simulink model "Crazyflie_Sim_R2025b"  (R2025b)
settings: Solver=ode15s  StopTime=20  RelTol=1e-5
InitFcn:
  | Crazyflie_Param
values from neighbouring files (symbols this model uses):
  g = 9.80665    [Crazyflie_Param.m]
  Ix_drone = 2.934e-5    (= 2.934e-05)    [Crazyflie_Param.m]
  Iy_drone = 4.981e-5    (= 4.981e-05)    [Crazyflie_Param.m]
  Iz_drone = 7.646e-5    (= 7.646e-05)    [Crazyflie_Param.m]
  J = 1/12*m*(0.051^2+0.005^2)    (= 7.878e-08)    [Crazyflie_Param.m]
  kq = 0.006    [Crazyflie_Param.m]
  l1 = 4.445    [Crazyflie_Param.m]
  m = 0.00036    [Crazyflie_Param.m]
  m_drone = 0.04316    [Crazyflie_Param.m]
undefined symbols (not defined in the file or in its folder): sigbuilder_block, X, Y, Z
libraries: sm_lib x57, slpidlib x19, nesl_utility x18, fl_lib x9
(part 2 of 4)

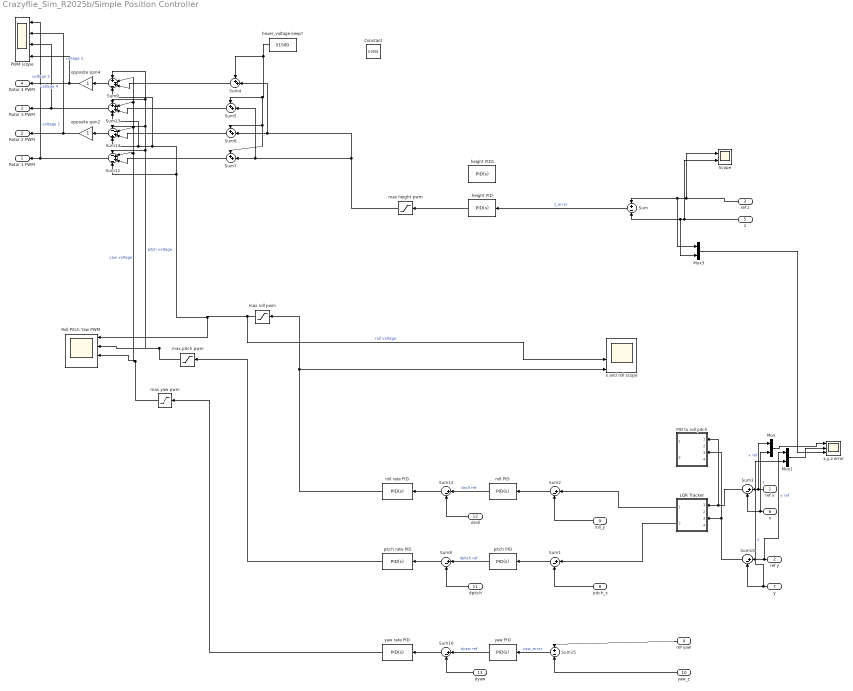
== system Crazyflie_Sim_R2025b/Simple Position Controller ==
  ref x : Inport
  ref y : Inport  Port=2
  ref z : Inport  Port=3
  ref yaw : Inport  Port=4
  z : Inport  Port=5
  x : Inport  Port=6
  y : Inport  Port=7
  pitch_x : Inport  Port=8
  roll_y : Inport  Port=9
  yaw_z : Inport  Port=10
  dpitch : Inport  Port=11
  droll : Inport  Port=12
  dyaw : Inport  Port=13
  Constant : Constant  Value=0.0001
  LQR Tracker : Subsystem
  Mux : Mux  Inputs=2
  Mux1 : Mux  Inputs=2
  Mux3 : Mux  Inputs=2
  PID to roll pitch : Subsystem
  PWM scope : Scope  NumInputPorts=4
      settings: ActiveDisplayYMinimum=30000  ActiveDisplayYMaximum=50000
  Roll Pitch Yaw PWM : Scope  NumInputPorts=4
      settings: ActiveDisplayYMinimum=-81918.75  ActiveDisplayYMaximum=81918.75
  Scope : Scope  NumInputPorts=2
      settings: ActiveDisplayYMinimum=-0.12883916669712672  ActiveDisplayYMaximum=1.1595525002741407  DataLoggingVariableName=ScopeData2
  Sum : Sum  Inputs=+-
  Sum{1..3,8,10,12,16} (7 alike) : Sum  Inputs=|+-
  Sum11 : Sum  Inputs=-++-
  Sum13 : Sum  Inputs=++++
  Sum14 : Sum  Inputs=--++
  Sum15 : Sum  Inputs=+-
  Sum{4..7} (4 alike) : Sum  Inputs=++|
  Sum9 : Sum  Inputs=+-+-
  height PID : slpidlib/PID Controller  Controller=PID  Form=Parallel  TimeDomain=Continuous-time  UseExternalTs=off  SampleTime=-1  IntegratorMethod=Forward Euler  FilterMethod=Forward Euler  ControllerParametersSource=internal  P=30000  I=100  UseKiTs=off  D=15000  UseExternalDerivativeSource=off  N=100  UseFilter=on  TunerSelectOption=Transfer Function Based (PID Tuner App)  ZeroCross=off  InitialConditionSource=internal  InitialConditionForIntegrator=0  InitialConditionForFilter=0  DifferentiatorICPrevScaledInput=0  ExternalReset=none  TrackingMode=off  Kt=1  LimitOutput=off  SatLimitsSource=internal  UpperSaturationLimit=inf  LowerSaturationLimit=-inf  LinearizeAsGain=on  AntiWindupMode=none  Kb=1  LimitIntegrator=off  UpperIntegratorSaturationLimit=inf  LowerIntegratorSaturationLimit=-inf  POutMin=[]  POutMax=[]  IOutMin=[]  IOutMax=[]  DOutMin=[]  DOutMax=[]  NOutMin=[]  NOutMax=[]  SumOutMin=[]  SumOutMax=[]  SaturationOutMin=[]  SaturationOutMax=[]  PParamMin=[]  PParamMax=[]  IParamMin=[]  IParamMax=[]  DParamMin=[]  DParamMax=[]  NParamMin=[]  NParamMax=[]  KbParamMin=[]  KbParamMax=[]  KtParamMin=[]  KtParamMax=[]  KbOutMin=[]  KbOutMax=[]  KtOutMin=[]  KtOutMax=[]  IntegratorOutMin=[]  IntegratorOutMax=[]  FilterOutMin=[]  FilterOutMax=[]  SumI1OutMin=[]  SumI1OutMax=[]  SumI2OutMin=[]  SumI2OutMax=[]  SumI3OutMin=[]  SumI3OutMax=[]  SumI4OutMin=[]  SumI4OutMax=[]  SumDOutMin=[]  SumDOutMax=[]  DifferentiatorOutMin=[]  DifferentiatorOutMax=[]  FilterDiffOutCoefMin=[]  FilterDiffOutCoefMax=[]  ReciprocalOutMin=[]  ReciprocalOutMax=[]  SumDenOutMin=[]  SumDenOutMax=[]  SumNumOutMin=[]  SumNumOutMax=[]  DivideOutMin=[]  DivideOutMax=[]  UdiffTsProdOutMin=[]  UdiffTsProdOutMax=[]  NTsProdOutMin=[]  NTsProdOutMax=[]  UintegralTsProdOutMin=[]  UintegralTsProdOutMax=[]  UngainTsProdOutMin=[]  UngainTsProdOutMax=[]  ClampingZeroOutDataTypeStr=Inherit: Inherit via back propagation  ClampingZeroOutMin=[]  ClampingZeroOutMax=[]  FilterDenConstantOutDataTypeStr=Inherit: Inherit via back propagation  FilterDenConstantOutMin=[]  FilterDenConstantOutMax=[]  PCopyOutDataTypeStr=Inherit: Inherit via back propagation  PCopyOutMin=[]  PCopyOutMax=[]  NCopyOutDataTypeStr=Inherit: Inherit via back propagation  NCopyOutMin=[]  NCopyOutMax=[]  IntegratorContinuousStateAttributes=''  IntegratorStateMustResolveToSignalObject=off  IntegratorRTWStateStorageClass=Auto  FilterContinuousStateAttributes=''  FilterStateMustResolveToSignalObject=off  FilterRTWStateStorageClass=Auto  ParallelPVariant=InternalParameters  IdealPVariant=Disabled  IVariant=InternalParameters  DVariant=InternalParameters  IntegratorVariant=Continuous  SatVariant=Disabled  AWVariant=Passthrough  PCopyVariant=Disabled  TRVariant=Disabled  FdbkBlocksVariant=Forward  IdealPFdbkVariant=Disabled  SatFdbkVariant=Disabled  DerivativeFilterVariant=ContFilter  NVariant=InternalParameters  NCopyVariant=Disabled  FilterICVariant=InternalICsFilter  IntegratorICVariant=InternalICs  ExternalResetVariant=Disabled  TRSumVariant=Passthrough  SumFdbkVariant=Disabled  SumVariant=Sum_PID  TsampFilterVariant=InternalTs  TsampNgainVariant=Passthrough  TsampIntegralVariant=Disabled_SignalSpec  ExternalSaturationOutDataTypeStr=Inherit: Same as second input  DerivativeSourceVariant=ErrorSignal  PreIntVariant=InternalPreInt
  height PID1 : slpidlib/PID Controller  Controller=PID  Form=Parallel  TimeDomain=Continuous-time  UseExternalTs=off  SampleTime=-1  IntegratorMethod=Forward Euler  FilterMethod=Forward Euler  ControllerParametersSource=internal  P=14649  I=0  UseKiTs=off  D=6252  UseExternalDerivativeSource=off  N=100  UseFilter=on  TunerSelectOption=Transfer Function Based (PID Tuner App)  InitialConditionSource=internal  InitialConditionForIntegrator=0  InitialConditionForFilter=0  DifferentiatorICPrevScaledInput=0  ExternalReset=none  TrackingMode=off  Kt=1  LimitOutput=off  SatLimitsSource=internal  UpperSaturationLimit=inf  LowerSaturationLimit=-inf  LinearizeAsGain=on  AntiWindupMode=none  Kb=1  LimitIntegrator=off  UpperIntegratorSaturationLimit=inf  LowerIntegratorSaturationLimit=-inf  POutMin=[]  POutMax=[]  IOutMin=[]  IOutMax=[]  DOutMin=[]  DOutMax=[]  NOutMin=[]  NOutMax=[]  SumOutMin=[]  SumOutMax=[]  SaturationOutMin=[]  SaturationOutMax=[]  PParamMin=[]  PParamMax=[]  IParamMin=[]  IParamMax=[]  DParamMin=[]  DParamMax=[]  NParamMin=[]  NParamMax=[]  KbParamMin=[]  KbParamMax=[]  KtParamMin=[]  KtParamMax=[]  KbOutMin=[]  KbOutMax=[]  KtOutMin=[]  KtOutMax=[]  IntegratorOutMin=[]  IntegratorOutMax=[]  FilterOutMin=[]  FilterOutMax=[]  SumI1OutMin=[]  SumI1OutMax=[]  SumI2OutMin=[]  SumI2OutMax=[]  SumI3OutMin=[]  SumI3OutMax=[]  SumI4OutMin=[]  SumI4OutMax=[]  SumDOutMin=[]  SumDOutMax=[]  DifferentiatorOutMin=[]  DifferentiatorOutMax=[]  FilterDiffOutCoefMin=[]  FilterDiffOutCoefMax=[]  ReciprocalOutMin=[]  ReciprocalOutMax=[]  SumDenOutMin=[]  SumDenOutMax=[]  SumNumOutMin=[]  SumNumOutMax=[]  DivideOutMin=[]  DivideOutMax=[]  UdiffTsProdOutMin=[]  UdiffTsProdOutMax=[]  NTsProdOutMin=[]  NTsProdOutMax=[]  UintegralTsProdOutMin=[]  UintegralTsProdOutMax=[]  UngainTsProdOutMin=[]  UngainTsProdOutMax=[]  ClampingZeroOutDataTypeStr=Inherit: Inherit via back propagation  ClampingZeroOutMin=[]  ClampingZeroOutMax=[]  FilterDenConstantOutDataTypeStr=Inherit: Inherit via back propagation  FilterDenConstantOutMin=[]  FilterDenConstantOutMax=[]  PCopyOutDataTypeStr=Inherit: Inherit via back propagation  PCopyOutMin=[]  PCopyOutMax=[]  NCopyOutDataTypeStr=Inherit: Inherit via back propagation  NCopyOutMin=[]  NCopyOutMax=[]  IntegratorContinuousStateAttributes=''  IntegratorStateMustResolveToSignalObject=off  IntegratorRTWStateStorageClass=Auto  FilterContinuousStateAttributes=''  FilterStateMustResolveToSignalObject=off  FilterRTWStateStorageClass=Auto  ParallelPVariant=InternalParameters  IdealPVariant=Disabled  IVariant=InternalParameters  DVariant=InternalParameters  IntegratorVariant=Continuous  SatVariant=Disabled  AWVariant=Passthrough  PCopyVariant=Disabled  TRVariant=Disabled  FdbkBlocksVariant=Forward  IdealPFdbkVariant=Disabled  SatFdbkVariant=Disabled  DerivativeFilterVariant=ContFilter  NVariant=InternalParameters  NCopyVariant=Disabled  FilterICVariant=InternalICsFilter  IntegratorICVariant=InternalICs  ExternalResetVariant=Disabled  TRSumVariant=Passthrough  SumFdbkVariant=Disabled  SumVariant=Sum_PID  TsampFilterVariant=InternalTs  TsampNgainVariant=Passthrough  TsampIntegralVariant=Disabled_SignalSpec  ExternalSaturationOutDataTypeStr=Inherit: Same as second input  DerivativeSourceVariant=ErrorSignal  PreIntVariant=InternalPreInt
  hover_voltage keep? : Constant  Value=51500
  max height pwm : Saturate  UpperLimit=30000  LowerLimit=-38000  ZeroCross=off
  max pitch pwm : Saturate  UpperLimit=10000  LowerLimit=-10000  ZeroCross=off
  max roll pwm : Saturate  UpperLimit=10000  LowerLimit=-10000  ZeroCross=off
  max yaw pwm : Saturate  UpperLimit=10000  LowerLimit=-10000  ZeroCross=off
  opposite spin2 : Gain
  opposite spin4 : Gain
  pitch PID : slpidlib/PID Controller  Controller=PID  Form=Parallel  TimeDomain=Continuous-time  UseExternalTs=off  SampleTime=-1  IntegratorMethod=Forward Euler  FilterMethod=Forward Euler  ControllerParametersSource=internal  P=6  I=3  UseKiTs=off  D=0  UseExternalDerivativeSource=off  N=100  UseFilter=on  TunerSelectOption=Transfer Function Based (PID Tuner App)  InitialConditionSource=internal  InitialConditionForIntegrator=0  InitialConditionForFilter=0  DifferentiatorICPrevScaledInput=0  ExternalReset=none  TrackingMode=off  Kt=1  LimitOutput=off  SatLimitsSource=internal  UpperSaturationLimit=inf  LowerSaturationLimit=-inf  LinearizeAsGain=on  AntiWindupMode=none  Kb=1  LimitIntegrator=off  UpperIntegratorSaturationLimit=inf  LowerIntegratorSaturationLimit=-inf  POutMin=[]  POutMax=[]  IOutMin=[]  IOutMax=[]  DOutMin=[]  DOutMax=[]  NOutMin=[]  NOutMax=[]  SumOutMin=[]  SumOutMax=[]  SaturationOutMin=[]  SaturationOutMax=[]  PParamMin=[]  PParamMax=[]  IParamMin=[]  IParamMax=[]  DParamMin=[]  DParamMax=[]  NParamMin=[]  NParamMax=[]  KbParamMin=[]  KbParamMax=[]  KtParamMin=[]  KtParamMax=[]  KbOutMin=[]  KbOutMax=[]  KtOutMin=[]  KtOutMax=[]  IntegratorOutMin=[]  IntegratorOutMax=[]  FilterOutMin=[]  FilterOutMax=[]  SumI1OutMin=[]  SumI1OutMax=[]  SumI2OutMin=[]  SumI2OutMax=[]  SumI3OutMin=[]  SumI3OutMax=[]  SumI4OutMin=[]  SumI4OutMax=[]  SumDOutMin=[]  SumDOutMax=[]  DifferentiatorOutMin=[]  DifferentiatorOutMax=[]  FilterDiffOutCoefMin=[]  FilterDiffOutCoefMax=[]  ReciprocalOutMin=[]  ReciprocalOutMax=[]  SumDenOutMin=[]  SumDenOutMax=[]  SumNumOutMin=[]  SumNumOutMax=[]  DivideOutMin=[]  DivideOutMax=[]  UdiffTsProdOutMin=[]  UdiffTsProdOutMax=[]  NTsProdOutMin=[]  NTsProdOutMax=[]  UintegralTsProdOutMin=[]  UintegralTsProdOutMax=[]  UngainTsProdOutMin=[]  UngainTsProdOutMax=[]  ClampingZeroOutDataTypeStr=Inherit: Inherit via back propagation  ClampingZeroOutMin=[]  ClampingZeroOutMax=[]  FilterDenConstantOutDataTypeStr=Inherit: Inherit via back propagation  FilterDenConstantOutMin=[]  FilterDenConstantOutMax=[]  PCopyOutDataTypeStr=Inherit: Inherit via back propagation  PCopyOutMin=[]  PCopyOutMax=[]  NCopyOutDataTypeStr=Inherit: Inherit via back propagation  NCopyOutMin=[]  NCopyOutMax=[]  IntegratorContinuousStateAttributes=''  IntegratorStateMustResolveToSignalObject=off  IntegratorRTWStateStorageClass=Auto  FilterContinuousStateAttributes=''  FilterStateMustResolveToSignalObject=off  FilterRTWStateStorageClass=Auto  ParallelPVariant=InternalParameters  IdealPVariant=Disabled  IVariant=InternalParameters  DVariant=InternalParameters  IntegratorVariant=Continuous  SatVariant=Disabled  AWVariant=Passthrough  PCopyVariant=Disabled  TRVariant=Disabled  FdbkBlocksVariant=Forward  IdealPFdbkVariant=Disabled  SatFdbkVariant=Disabled  DerivativeFilterVariant=ContFilter  NVariant=InternalParameters  NCopyVariant=Disabled  FilterICVariant=InternalICsFilter  IntegratorICVariant=InternalICs  ExternalResetVariant=Disabled  TRSumVariant=Passthrough  SumFdbkVariant=Disabled  SumVariant=Sum_PID  TsampFilterVariant=InternalTs  TsampNgainVariant=Passthrough  TsampIntegralVariant=Disabled_SignalSpec  ExternalSaturationOutDataTypeStr=Inherit: Same as second input  DerivativeSourceVariant=ErrorSignal  PreIntVariant=InternalPreInt
  pitch rate PID : slpidlib/PID Controller  Controller=PID  Form=Parallel  TimeDomain=Continuous-time  UseExternalTs=off  SampleTime=-1  IntegratorMethod=Forward Euler  FilterMethod=Forward Euler  ControllerParametersSource=internal  P=250*3.1  I=500*3.1  UseKiTs=off  D=2.5*3.1  UseExternalDerivativeSource=off  N=100  UseFilter=on  TunerSelectOption=Transfer Function Based (PID Tuner App)  InitialConditionSource=internal  InitialConditionForIntegrator=0  InitialConditionForFilter=0  DifferentiatorICPrevScaledInput=0  ExternalReset=none  TrackingMode=off  Kt=1  LimitOutput=off  SatLimitsSource=internal  UpperSaturationLimit=inf  LowerSaturationLimit=-inf  LinearizeAsGain=on  AntiWindupMode=none  Kb=1  LimitIntegrator=off  UpperIntegratorSaturationLimit=inf  LowerIntegratorSaturationLimit=-inf  POutMin=[]  POutMax=[]  IOutMin=[]  IOutMax=[]  DOutMin=[]  DOutMax=[]  NOutMin=[]  NOutMax=[]  SumOutMin=[]  SumOutMax=[]  SaturationOutMin=[]  SaturationOutMax=[]  PParamMin=[]  PParamMax=[]  IParamMin=[]  IParamMax=[]  DParamMin=[]  DParamMax=[]  NParamMin=[]  NParamMax=[]  KbParamMin=[]  KbParamMax=[]  KtParamMin=[]  KtParamMax=[]  KbOutMin=[]  KbOutMax=[]  KtOutMin=[]  KtOutMax=[]  IntegratorOutMin=[]  IntegratorOutMax=[]  FilterOutMin=[]  FilterOutMax=[]  SumI1OutMin=[]  SumI1OutMax=[]  SumI2OutMin=[]  SumI2OutMax=[]  SumI3OutMin=[]  SumI3OutMax=[]  SumI4OutMin=[]  SumI4OutMax=[]  SumDOutMin=[]  SumDOutMax=[]  DifferentiatorOutMin=[]  DifferentiatorOutMax=[]  FilterDiffOutCoefMin=[]  FilterDiffOutCoefMax=[]  ReciprocalOutMin=[]  ReciprocalOutMax=[]  SumDenOutMin=[]  SumDenOutMax=[]  SumNumOutMin=[]  SumNumOutMax=[]  DivideOutMin=[]  DivideOutMax=[]  UdiffTsProdOutMin=[]  UdiffTsProdOutMax=[]  NTsProdOutMin=[]  NTsProdOutMax=[]  UintegralTsProdOutMin=[]  UintegralTsProdOutMax=[]  UngainTsProdOutMin=[]  UngainTsProdOutMax=[]  ClampingZeroOutDataTypeStr=Inherit: Inherit via back propagation  ClampingZeroOutMin=[]  ClampingZeroOutMax=[]  FilterDenConstantOutDataTypeStr=Inherit: Inherit via back propagation  FilterDenConstantOutMin=[]  FilterDenConstantOutMax=[]  PCopyOutDataTypeStr=Inherit: Inherit via back propagation  PCopyOutMin=[]  PCopyOutMax=[]  NCopyOutDataTypeStr=Inherit: Inherit via back propagation  NCopyOutMin=[]  NCopyOutMax=[]  IntegratorContinuousStateAttributes=''  IntegratorStateMustResolveToSignalObject=off  IntegratorRTWStateStorageClass=Auto  FilterContinuousStateAttributes=''  FilterStateMustResolveToSignalObject=off  FilterRTWStateStorageClass=Auto  ParallelPVariant=InternalParameters  IdealPVariant=Disabled  IVariant=InternalParameters  DVariant=InternalParameters  IntegratorVariant=Continuous  SatVariant=Disabled  AWVariant=Passthrough  PCopyVariant=Disabled  TRVariant=Disabled  FdbkBlocksVariant=Forward  IdealPFdbkVariant=Disabled  SatFdbkVariant=Disabled  DerivativeFilterVariant=ContFilter  NVariant=InternalParameters  NCopyVariant=Disabled  FilterICVariant=InternalICsFilter  IntegratorICVariant=InternalICs  ExternalResetVariant=Disabled  TRSumVariant=Passthrough  SumFdbkVariant=Disabled  SumVariant=Sum_PID  TsampFilterVariant=InternalTs  TsampNgainVariant=Passthrough  TsampIntegralVariant=Disabled_SignalSpec  ExternalSaturationOutDataTypeStr=Inherit: Same as second input  DerivativeSourceVariant=ErrorSignal  PreIntVariant=InternalPreInt
  roll PID : slpidlib/PID Controller  Controller=PID  Form=Parallel  TimeDomain=Continuous-time  UseExternalTs=off  SampleTime=-1  IntegratorMethod=Forward Euler  FilterMethod=Forward Euler  ControllerParametersSource=internal  P=6  I=3  UseKiTs=off  D=0  UseExternalDerivativeSource=off  N=100  UseFilter=on  TunerSelectOption=Transfer Function Based (PID Tuner App)  InitialConditionSource=internal  InitialConditionForIntegrator=0  InitialConditionForFilter=0  DifferentiatorICPrevScaledInput=0  ExternalReset=none  TrackingMode=off  Kt=1  LimitOutput=off  SatLimitsSource=internal  UpperSaturationLimit=inf  LowerSaturationLimit=-inf  LinearizeAsGain=on  AntiWindupMode=none  Kb=1  LimitIntegrator=off  UpperIntegratorSaturationLimit=inf  LowerIntegratorSaturationLimit=-inf  POutMin=[]  POutMax=[]  IOutMin=[]  IOutMax=[]  DOutMin=[]  DOutMax=[]  NOutMin=[]  NOutMax=[]  SumOutMin=[]  SumOutMax=[]  SaturationOutMin=[]  SaturationOutMax=[]  PParamMin=[]  PParamMax=[]  IParamMin=[]  IParamMax=[]  DParamMin=[]  DParamMax=[]  NParamMin=[]  NParamMax=[]  KbParamMin=[]  KbParamMax=[]  KtParamMin=[]  KtParamMax=[]  KbOutMin=[]  KbOutMax=[]  KtOutMin=[]  KtOutMax=[]  IntegratorOutMin=[]  IntegratorOutMax=[]  FilterOutMin=[]  FilterOutMax=[]  SumI1OutMin=[]  SumI1OutMax=[]  SumI2OutMin=[]  SumI2OutMax=[]  SumI3OutMin=[]  SumI3OutMax=[]  SumI4OutMin=[]  SumI4OutMax=[]  SumDOutMin=[]  SumDOutMax=[]  DifferentiatorOutMin=[]  DifferentiatorOutMax=[]  FilterDiffOutCoefMin=[]  FilterDiffOutCoefMax=[]  ReciprocalOutMin=[]  ReciprocalOutMax=[]  SumDenOutMin=[]  SumDenOutMax=[]  SumNumOutMin=[]  SumNumOutMax=[]  DivideOutMin=[]  DivideOutMax=[]  UdiffTsProdOutMin=[]  UdiffTsProdOutMax=[]  NTsProdOutMin=[]  NTsProdOutMax=[]  UintegralTsProdOutMin=[]  UintegralTsProdOutMax=[]  UngainTsProdOutMin=[]  UngainTsProdOutMax=[]  ClampingZeroOutDataTypeStr=Inherit: Inherit via back propagation  ClampingZeroOutMin=[]  ClampingZeroOutMax=[]  FilterDenConstantOutDataTypeStr=Inherit: Inherit via back propagation  FilterDenConstantOutMin=[]  FilterDenConstantOutMax=[]  PCopyOutDataTypeStr=Inherit: Inherit via back propagation  PCopyOutMin=[]  PCopyOutMax=[]  NCopyOutDataTypeStr=Inherit: Inherit via back propagation  NCopyOutMin=[]  NCopyOutMax=[]  IntegratorContinuousStateAttributes=''  IntegratorStateMustResolveToSignalObject=off  IntegratorRTWStateStorageClass=Auto  FilterContinuousStateAttributes=''  FilterStateMustResolveToSignalObject=off  FilterRTWStateStorageClass=Auto  ParallelPVariant=InternalParameters  IdealPVariant=Disabled  IVariant=InternalParameters  DVariant=InternalParameters  IntegratorVariant=Continuous  SatVariant=Disabled  AWVariant=Passthrough  PCopyVariant=Disabled  TRVariant=Disabled  FdbkBlocksVariant=Forward  IdealPFdbkVariant=Disabled  SatFdbkVariant=Disabled  DerivativeFilterVariant=ContFilter  NVariant=InternalParameters  NCopyVariant=Disabled  FilterICVariant=InternalICsFilter  IntegratorICVariant=InternalICs  ExternalResetVariant=Disabled  TRSumVariant=Passthrough  SumFdbkVariant=Disabled  SumVariant=Sum_PID  TsampFilterVariant=InternalTs  TsampNgainVariant=Passthrough  TsampIntegralVariant=Disabled_SignalSpec  ExternalSaturationOutDataTypeStr=Inherit: Same as second input  DerivativeSourceVariant=ErrorSignal  PreIntVariant=InternalPreInt
  roll rate PID : slpidlib/PID Controller  Controller=PID  Form=Parallel  TimeDomain=Continuous-time  UseExternalTs=off  SampleTime=-1  IntegratorMethod=Forward Euler  FilterMethod=Forward Euler  ControllerParametersSource=internal  P=250*3.1  I=500*3.1  UseKiTs=off  D=2.5*3.1  UseExternalDerivativeSource=off  N=100  UseFilter=on  TunerSelectOption=Transfer Function Based (PID Tuner App)  InitialConditionSource=internal  InitialConditionForIntegrator=0  InitialConditionForFilter=0  DifferentiatorICPrevScaledInput=0  ExternalReset=none  TrackingMode=off  Kt=1  LimitOutput=off  SatLimitsSource=internal  UpperSaturationLimit=inf  LowerSaturationLimit=-inf  LinearizeAsGain=on  AntiWindupMode=none  Kb=1  LimitIntegrator=off  UpperIntegratorSaturationLimit=inf  LowerIntegratorSaturationLimit=-inf  POutMin=[]  POutMax=[]  IOutMin=[]  IOutMax=[]  DOutMin=[]  DOutMax=[]  NOutMin=[]  NOutMax=[]  SumOutMin=[]  SumOutMax=[]  SaturationOutMin=[]  SaturationOutMax=[]  PParamMin=[]  PParamMax=[]  IParamMin=[]  IParamMax=[]  DParamMin=[]  DParamMax=[]  NParamMin=[]  NParamMax=[]  KbParamMin=[]  KbParamMax=[]  KtParamMin=[]  KtParamMax=[]  KbOutMin=[]  KbOutMax=[]  KtOutMin=[]  KtOutMax=[]  IntegratorOutMin=[]  IntegratorOutMax=[]  FilterOutMin=[]  FilterOutMax=[]  SumI1OutMin=[]  SumI1OutMax=[]  SumI2OutMin=[]  SumI2OutMax=[]  SumI3OutMin=[]  SumI3OutMax=[]  SumI4OutMin=[]  SumI4OutMax=[]  SumDOutMin=[]  SumDOutMax=[]  DifferentiatorOutMin=[]  DifferentiatorOutMax=[]  FilterDiffOutCoefMin=[]  FilterDiffOutCoefMax=[]  ReciprocalOutMin=[]  ReciprocalOutMax=[]  SumDenOutMin=[]  SumDenOutMax=[]  SumNumOutMin=[]  SumNumOutMax=[]  DivideOutMin=[]  DivideOutMax=[]  UdiffTsProdOutMin=[]  UdiffTsProdOutMax=[]  NTsProdOutMin=[]  NTsProdOutMax=[]  UintegralTsProdOutMin=[]  UintegralTsProdOutMax=[]  UngainTsProdOutMin=[]  UngainTsProdOutMax=[]  ClampingZeroOutDataTypeStr=Inherit: Inherit via back propagation  ClampingZeroOutMin=[]  ClampingZeroOutMax=[]  FilterDenConstantOutDataTypeStr=Inherit: Inherit via back propagation  FilterDenConstantOutMin=[]  FilterDenConstantOutMax=[]  PCopyOutDataTypeStr=Inherit: Inherit via back propagation  PCopyOutMin=[]  PCopyOutMax=[]  NCopyOutDataTypeStr=Inherit: Inherit via back propagation  NCopyOutMin=[]  NCopyOutMax=[]  IntegratorContinuousStateAttributes=''  IntegratorStateMustResolveToSignalObject=off  IntegratorRTWStateStorageClass=Auto  FilterContinuousStateAttributes=''  FilterStateMustResolveToSignalObject=off  FilterRTWStateStorageClass=Auto  ParallelPVariant=InternalParameters  IdealPVariant=Disabled  IVariant=InternalParameters  DVariant=InternalParameters  IntegratorVariant=Continuous  SatVariant=Disabled  AWVariant=Passthrough  PCopyVariant=Disabled  TRVariant=Disabled  FdbkBlocksVariant=Forward  IdealPFdbkVariant=Disabled  SatFdbkVariant=Disabled  DerivativeFilterVariant=ContFilter  NVariant=InternalParameters  NCopyVariant=Disabled  FilterICVariant=InternalICsFilter  IntegratorICVariant=InternalICs  ExternalResetVariant=Disabled  TRSumVariant=Passthrough  SumFdbkVariant=Disabled  SumVariant=Sum_PID  TsampFilterVariant=InternalTs  TsampNgainVariant=Passthrough  TsampIntegralVariant=Disabled_SignalSpec  ExternalSaturationOutDataTypeStr=Inherit: Same as second input  DerivativeSourceVariant=ErrorSignal  PreIntVariant=InternalPreInt
  "x and roll scope " : Scope  NumInputPorts=4
      settings: ActiveDisplayYMinimum=-11.1433  ActiveDisplayYMaximum=1.32628  DataLoggingVariableName=ScopeData3
  x,y,z error : Scope  NumInputPorts=3
      settings: ActiveDisplayYMinimum=-0.13989491710179006  ActiveDisplayYMaximum=1.25875136013476  DataLoggingVariableName=ScopeData2
  yaw PID : slpidlib/PID Controller  Controller=PID  Form=Parallel  TimeDomain=Continuous-time  UseExternalTs=off  SampleTime=-1  IntegratorMethod=Forward Euler  FilterMethod=Forward Euler  ControllerParametersSource=internal  P=6  I=1  UseKiTs=off  D=0.35  UseExternalDerivativeSource=off  N=100  UseFilter=on  TunerSelectOption=Transfer Function Based (PID Tuner App)  InitialConditionSource=internal  InitialConditionForIntegrator=0  InitialConditionForFilter=0  DifferentiatorICPrevScaledInput=0  ExternalReset=none  TrackingMode=off  Kt=1  LimitOutput=off  SatLimitsSource=internal  UpperSaturationLimit=inf  LowerSaturationLimit=-inf  LinearizeAsGain=on  AntiWindupMode=none  Kb=1  LimitIntegrator=off  UpperIntegratorSaturationLimit=inf  LowerIntegratorSaturationLimit=-inf  POutMin=[]  POutMax=[]  IOutMin=[]  IOutMax=[]  DOutMin=[]  DOutMax=[]  NOutMin=[]  NOutMax=[]  SumOutMin=[]  SumOutMax=[]  SaturationOutMin=[]  SaturationOutMax=[]  PParamMin=[]  PParamMax=[]  IParamMin=[]  IParamMax=[]  DParamMin=[]  DParamMax=[]  NParamMin=[]  NParamMax=[]  KbParamMin=[]  KbParamMax=[]  KtParamMin=[]  KtParamMax=[]  KbOutMin=[]  KbOutMax=[]  KtOutMin=[]  KtOutMax=[]  IntegratorOutMin=[]  IntegratorOutMax=[]  FilterOutMin=[]  FilterOutMax=[]  SumI1OutMin=[]  SumI1OutMax=[]  SumI2OutMin=[]  SumI2OutMax=[]  SumI3OutMin=[]  SumI3OutMax=[]  SumI4OutMin=[]  SumI4OutMax=[]  SumDOutMin=[]  SumDOutMax=[]  DifferentiatorOutMin=[]  DifferentiatorOutMax=[]  FilterDiffOutCoefMin=[]  FilterDiffOutCoefMax=[]  ReciprocalOutMin=[]  ReciprocalOutMax=[]  SumDenOutMin=[]  SumDenOutMax=[]  SumNumOutMin=[]  SumNumOutMax=[]  DivideOutMin=[]  DivideOutMax=[]  UdiffTsProdOutMin=[]  UdiffTsProdOutMax=[]  NTsProdOutMin=[]  NTsProdOutMax=[]  UintegralTsProdOutMin=[]  UintegralTsProdOutMax=[]  UngainTsProdOutMin=[]  UngainTsProdOutMax=[]  ClampingZeroOutDataTypeStr=Inherit: Inherit via back propagation  ClampingZeroOutMin=[]  ClampingZeroOutMax=[]  FilterDenConstantOutDataTypeStr=Inherit: Inherit via back propagation  FilterDenConstantOutMin=[]  FilterDenConstantOutMax=[]  PCopyOutDataTypeStr=Inherit: Inherit via back propagation  PCopyOutMin=[]  PCopyOutMax=[]  NCopyOutDataTypeStr=Inherit: Inherit via back propagation  NCopyOutMin=[]  NCopyOutMax=[]  IntegratorContinuousStateAttributes=''  IntegratorStateMustResolveToSignalObject=off  IntegratorRTWStateStorageClass=Auto  FilterContinuousStateAttributes=''  FilterStateMustResolveToSignalObject=off  FilterRTWStateStorageClass=Auto  ParallelPVariant=InternalParameters  IdealPVariant=Disabled  IVariant=InternalParameters  DVariant=InternalParameters  IntegratorVariant=Continuous  SatVariant=Disabled  AWVariant=Passthrough  PCopyVariant=Disabled  TRVariant=Disabled  FdbkBlocksVariant=Forward  IdealPFdbkVariant=Disabled  SatFdbkVariant=Disabled  DerivativeFilterVariant=ContFilter  NVariant=InternalParameters  NCopyVariant=Disabled  FilterICVariant=InternalICsFilter  IntegratorICVariant=InternalICs  ExternalResetVariant=Disabled  TRSumVariant=Passthrough  SumFdbkVariant=Disabled  SumVariant=Sum_PID  TsampFilterVariant=InternalTs  TsampNgainVariant=Passthrough  TsampIntegralVariant=Disabled_SignalSpec  ExternalSaturationOutDataTypeStr=Inherit: Same as second input  DerivativeSourceVariant=ErrorSignal  PreIntVariant=InternalPreInt
  yaw rate PID : slpidlib/PID Controller  Controller=PID  Form=Parallel  TimeDomain=Continuous-time  UseExternalTs=off  SampleTime=-1  IntegratorMethod=Forward Euler  FilterMethod=Forward Euler  ControllerParametersSource=internal  P=120*3.1  I=16.7*3.1  UseKiTs=off  D=0  UseExternalDerivativeSource=off  N=100  UseFilter=on  TunerSelectOption=Transfer Function Based (PID Tuner App)  InitialConditionSource=internal  InitialConditionForIntegrator=0  InitialConditionForFilter=0  DifferentiatorICPrevScaledInput=0  ExternalReset=none  TrackingMode=off  Kt=1  LimitOutput=off  SatLimitsSource=internal  UpperSaturationLimit=inf  LowerSaturationLimit=-inf  LinearizeAsGain=on  AntiWindupMode=none  Kb=1  LimitIntegrator=off  UpperIntegratorSaturationLimit=inf  LowerIntegratorSaturationLimit=-inf  POutMin=[]  POutMax=[]  IOutMin=[]  IOutMax=[]  DOutMin=[]  DOutMax=[]  NOutMin=[]  NOutMax=[]  SumOutMin=[]  SumOutMax=[]  SaturationOutMin=[]  SaturationOutMax=[]  PParamMin=[]  PParamMax=[]  IParamMin=[]  IParamMax=[]  DParamMin=[]  DParamMax=[]  NParamMin=[]  NParamMax=[]  KbParamMin=[]  KbParamMax=[]  KtParamMin=[]  KtParamMax=[]  KbOutMin=[]  KbOutMax=[]  KtOutMin=[]  KtOutMax=[]  IntegratorOutMin=[]  IntegratorOutMax=[]  FilterOutMin=[]  FilterOutMax=[]  SumI1OutMin=[]  SumI1OutMax=[]  SumI2OutMin=[]  SumI2OutMax=[]  SumI3OutMin=[]  SumI3OutMax=[]  SumI4OutMin=[]  SumI4OutMax=[]  SumDOutMin=[]  SumDOutMax=[]  DifferentiatorOutMin=[]  DifferentiatorOutMax=[]  FilterDiffOutCoefMin=[]  FilterDiffOutCoefMax=[]  ReciprocalOutMin=[]  ReciprocalOutMax=[]  SumDenOutMin=[]  SumDenOutMax=[]  SumNumOutMin=[]  SumNumOutMax=[]  DivideOutMin=[]  DivideOutMax=[]  UdiffTsProdOutMin=[]  UdiffTsProdOutMax=[]  NTsProdOutMin=[]  NTsProdOutMax=[]  UintegralTsProdOutMin=[]  UintegralTsProdOutMax=[]  UngainTsProdOutMin=[]  UngainTsProdOutMax=[]  ClampingZeroOutDataTypeStr=Inherit: Inherit via back propagation  ClampingZeroOutMin=[]  ClampingZeroOutMax=[]  FilterDenConstantOutDataTypeStr=Inherit: Inherit via back propagation  FilterDenConstantOutMin=[]  FilterDenConstantOutMax=[]  PCopyOutDataTypeStr=Inherit: Inherit via back propagation  PCopyOutMin=[]  PCopyOutMax=[]  NCopyOutDataTypeStr=Inherit: Inherit via back propagation  NCopyOutMin=[]  NCopyOutMax=[]  IntegratorContinuousStateAttributes=''  IntegratorStateMustResolveToSignalObject=off  IntegratorRTWStateStorageClass=Auto  FilterContinuousStateAttributes=''  FilterStateMustResolveToSignalObject=off  FilterRTWStateStorageClass=Auto  ParallelPVariant=InternalParameters  IdealPVariant=Disabled  IVariant=InternalParameters  DVariant=InternalParameters  IntegratorVariant=Continuous  SatVariant=Disabled  AWVariant=Passthrough  PCopyVariant=Disabled  TRVariant=Disabled  FdbkBlocksVariant=Forward  IdealPFdbkVariant=Disabled  SatFdbkVariant=Disabled  DerivativeFilterVariant=ContFilter  NVariant=InternalParameters  NCopyVariant=Disabled  FilterICVariant=InternalICsFilter  IntegratorICVariant=InternalICs  ExternalResetVariant=Disabled  TRSumVariant=Passthrough  SumFdbkVariant=Disabled  SumVariant=Sum_PID  TsampFilterVariant=InternalTs  TsampNgainVariant=Passthrough  TsampIntegralVariant=Disabled_SignalSpec  ExternalSaturationOutDataTypeStr=Inherit: Same as second input  DerivativeSourceVariant=ErrorSignal  PreIntVariant=InternalPreInt
  Rotor 1 PWM : Outport
  Rotor 2 PWM : Outport  Port=2
  Rotor 3 PWM : Outport  Port=3
  Rotor 4 PWM : Outport  Port=4
  wires:
  hover_voltage keep?/1 -> Sum4/1, Sum7/1, Sum6/1, Sum5/1
  Sum13/1 -> PWM scope/3, Rotor 3 PWM/1  "voltage 3"
  Sum11/1 -> Rotor 1 PWM/1, PWM scope/1  "voltage 1"
  Sum4/1 -> Sum9/3
  Sum6/1 -> Sum14/3
  opposite spin4/1 -> Rotor 4 PWM/1, PWM scope/4  "voltage 4"
  opposite spin2/1 -> PWM scope/2, Rotor 2 PWM/1  "voltage 2"
  ref z/1 -> Mux3/1, Sum/1, Scope/1
  z/1 -> Mux3/2, Sum/2, Scope/2
  Sum/1 -> height PID/1  "z_error"
  max roll pwm/1 -> Sum11/4, Sum14/4, Sum13/4, Sum9/4, Roll Pitch Yaw PWM/1, "x and roll scope "/3  "roll voltage"
  roll PID/1 -> Sum12/1  "droll ref"
  droll/1 -> Sum12/2
  Sum12/1 -> roll rate PID/1
  roll rate PID/1 -> max roll pwm/1, "x and roll scope "/4
  Sum8/1 -> pitch rate PID/1
  dpitch/1 -> Sum8/2
  pitch PID/1 -> Sum8/1  "dpitch ref"
  Sum5/1 -> Sum13/3
  Sum14/1 -> opposite spin2/1
  Sum9/1 -> opposite spin4/1
  Sum7/1 -> Sum11/3
  pitch rate PID/1 -> max pitch pwm/1
  max pitch pwm/1 -> Sum11/1, Sum14/1, Sum13/1, Sum9/1, Roll Pitch Yaw PWM/2  "pitch voltage"
  yaw rate PID/1 -> max yaw pwm/1
  ref yaw/1 -> Sum15/1
  yaw_z/1 -> Sum15/2
  Sum15/1 -> yaw PID/1  "yaw_error"
  yaw PID/1 -> Sum16/1  "dyaw ref"
  dyaw/1 -> Sum16/2
  Sum16/1 -> yaw rate PID/1
  max yaw pwm/1 -> Sum11/2, Sum14/2, Sum13/2, Sum9/2, Roll Pitch Yaw PWM/3  "yaw voltage"
  height PID/1 -> max height pwm/1
  Sum1/1 -> pitch PID/1
  pitch_x/1 -> Sum1/2
  Sum2/1 -> roll PID/1
  roll_y/1 -> Sum2/2
  ref x/1 -> Mux/1, Sum3/1  "x ref"
  x/1 -> Mux/2, Sum3/2  "x"
  ref y/1 -> Mux1/1, Sum10/1  "y ref"
  y/1 -> Mux1/2, Sum10/2  "y"
  Sum10/1 -> LQR Tracker/3(y error), PID to roll pitch/3(y error)
  Sum3/1 -> PID to roll pitch/1(x error), LQR Tracker/1(x error)
  LQR Tracker/1(roll ref) -> Sum2/1
  LQR Tracker/2(pitch ref) -> Sum1/1
  Mux/1 -> x,y,z error/1
  Mux1/1 -> x,y,z error/2
  max height pwm/1 -> Sum7/2, Sum5/2, Sum6/2, Sum4/2
  Mux3/1 -> x,y,z error/3

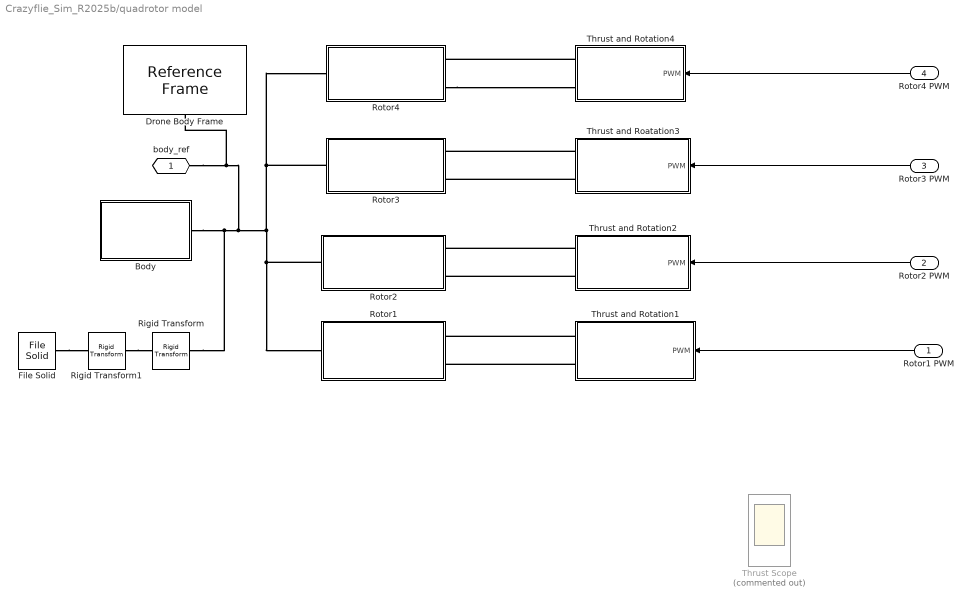
== system Crazyflie_Sim_R2025b/quadrotor model ==
  Rotor1 PWM : Inport
  Rotor2 PWM : Inport  Port=2
  Rotor3 PWM : Inport  Port=3
  Rotor4 PWM : Inport  Port=4
  Body : Subsystem
  Drone Body Frame : sm_lib/Frames and Transforms/Reference Frame
  File Solid : sm_lib/Body Elements/File Solid  ExtGeomFileName=C:\Users\lapsi\Documents\Work\Assignments\24-774\Project\CAD\Modified Crazyflie.step  UnitType=Custom  ExtGeomFileUnits=mm  StepReaderType=HEX  ExportConvexHullGeometry=off  InertiaType=PointMass  BasedOnType=DensityFromFile  Density=1000  DensityUnits=kg/m^3  Mass=0  MassUnits=kg  CenterOfMass=[0 0 0]  CenterOfMassUnits=m  MomentsOfInertia=[1 1 1]  MomentsOfInertiaUnits=kg*m^2  ProductsOfInertia=[0 0 0]  ProductsOfInertiaUnits=kg*m^2  GraphicType=FromGeometry  MarkerShape=Sphere  MarkerSize=10  GraphicVisPropType=AdvancedVisualProperties  GraphicDiffuseColor=[0.5 0.5 0.5]  GraphicOpacity=1  GraphicSpecularColor=[0.5 0.5 0.5 1.0]  GraphicAmbientColor=[0.15 0.15 0.15 1.0]  GraphicEmissiveColor=[0.0 0.0 0.0 1.0]  GraphicShininess=75  DoExposeReferenceFrame=on  SerializedFrames=<Frames/>
  Rigid Transform : sm_lib/Frames and Transforms/Rigid Transform  RotationMethod=StandardAxis  FollAlignAxisA=+X  BaseAlignAxisA=+Y  FollAlignAxisB=+Y  BaseAlignAxisB=+Z  RotationStandardAxis=+Z  RotationAngle=45  RotationAngleUnits=deg  RotationArbitraryAxis=[0 0 1]  RotationSequenceAxes=FollowerAxes  RotationSequence=XYX  RotationSequenceAngles=[0 0 0]  RotationSequenceAnglesUnits=deg  RotationMatrix=[1 0 0;0 1 0;0 0 1]  Quaternion=[1 0 0 0]  TranslationMethod=None  TranslationCartesianOffset=[0 0 0]  TranslationCartesianOffsetUnits=m  TranslationStandardAxis=+Z  TranslationStandardOffset=0  TranslationStandardOffsetUnits=m  TranslationROffset=0  TranslationROffsetUnits=m  TranslationThetaOffset=0  TranslationThetaOffsetUnits=deg  TranslationZOffset=0  TranslationZOffsetUnits=m
  Rigid Transform1 : sm_lib/Frames and Transforms/Rigid Transform  RotationMethod=StandardAxis  FollAlignAxisA=+X  BaseAlignAxisA=+Y  FollAlignAxisB=+Y  BaseAlignAxisB=+Z  RotationStandardAxis=+X  RotationAngle=180  RotationAngleUnits=deg  RotationArbitraryAxis=[0 0 1]  RotationSequenceAxes=FollowerAxes  RotationSequence=XYX  RotationSequenceAngles=[0 0 0]  RotationSequenceAnglesUnits=deg  RotationMatrix=[1 0 0;0 1 0;0 0 1]  Quaternion=[1 0 0 0]  TranslationMethod=None  TranslationCartesianOffset=[0 0 0]  TranslationCartesianOffsetUnits=m  TranslationStandardAxis=+Z  TranslationStandardOffset=0  TranslationStandardOffsetUnits=m  TranslationROffset=0  TranslationROffsetUnits=m  TranslationThetaOffset=0  TranslationThetaOffsetUnits=deg  TranslationZOffset=0  TranslationZOffsetUnits=m
  Rotor1 : Subsystem
  Rotor2 : Subsystem
  Rotor3 : Subsystem
  Rotor4 : Subsystem
  Thrust Scope : Scope  Commented=on  NumInputPorts=4
      settings: ActiveDisplayYMinimum=-1  ActiveDisplayYMaximum=1  DataLoggingVariableName=ScopeData2
  Thrust and Roatation3 : Subsystem
  Thrust and Rotation1 : Subsystem
  Thrust and Rotation2 : Subsystem
  Thrust and Rotation4 : Subsystem
  body_ref : PMIOPort  Side=Right
  wires:
  Rotor1 PWM/1 -> Thrust and Rotation1/1(PWM)
  Rotor2 PWM/1 -> Thrust and Rotation2/1(PWM)
  Rotor3 PWM/1 -> Thrust and Roatation3/1(PWM)
  Rotor4 PWM/1 -> Thrust and Rotation4/1(PWM)
  connections:
  Body/RConn1 -- Rigid Transform/RConn1 -- Rotor1/RConn1 -- Rotor2/LConn1 -- Rotor3/LConn1 -- Rotor4/LConn1 -- body_ref/RConn1 -- Drone Body Frame/RConn1
  Thrust and Rotation1/RConn1 -- Rotor1/LConn1
  Thrust and Rotation2/RConn1 -- Rotor2/RConn1
  Thrust and Rotation2/RConn2 -- Rotor2/RConn2
  Thrust and Roatation3/RConn1 -- Rotor3/RConn1
  Thrust and Rotation4/RConn1 -- Rotor4/RConn1
  File Solid/RConn1 -- Rigid Transform1/LConn1
  Rigid Transform1/RConn1 -- Rigid Transform/LConn1
  Thrust and Rotation1/RConn2 -- Rotor1/LConn2
  Thrust and Roatation3/RConn2 -- Rotor3/RConn2
  Rotor4/RConn2 -- Thrust and Rotation4/RConn2

== system Crazyflie_Sim_R2025b/6dof joint/Drone Reference Frame z-down,  + ==
  x +90 : sm_lib/Frames and Transforms/Rigid Transform  RotationMethod=StandardAxis  FollAlignAxisA=+X  BaseAlignAxisA=+Y  FollAlignAxisB=+Y  BaseAlignAxisB=+Z  RotationStandardAxis=+X  RotationAngle=90  RotationAngleUnits=deg  RotationArbitraryAxis=[0 0 1]  RotationSequenceAxes=FollowerAxes  RotationSequence=XYX  RotationSequenceAngles=[0 0 0]  RotationSequenceAnglesUnits=deg  RotationMatrix=[1 0 0; 0 1 0; 0 0 1]  Quaternion=[1 0 0 0]  TranslationMethod=None  TranslationCartesianOffset=[0 0 0]  TranslationCartesianOffsetUnits=m  TranslationStandardAxis=+Z  TranslationStandardOffset=0  TranslationStandardOffsetUnits=m  TranslationROffset=0  TranslationROffsetUnits=m  TranslationThetaOffset=0  TranslationThetaOffsetUnits=deg  TranslationZOffset=0  TranslationZOffsetUnits=m
  y -90 : sm_lib/Frames and Transforms/Rigid Transform  RotationMethod=StandardAxis  FollAlignAxisA=+X  BaseAlignAxisA=+Y  FollAlignAxisB=+Y  BaseAlignAxisB=+Z  RotationStandardAxis=+Y  RotationAngle=-90  RotationAngleUnits=deg  RotationArbitraryAxis=[0 0 1]  RotationSequenceAxes=FollowerAxes  RotationSequence=XYX  RotationSequenceAngles=[0 0 0]  RotationSequenceAnglesUnits=deg  RotationMatrix=[1 0 0; 0 1 0; 0 0 1]  Quaternion=[1 0 0 0]  TranslationMethod=None  TranslationCartesianOffset=[0 0 0]  TranslationCartesianOffsetUnits=m  TranslationStandardAxis=+Z  TranslationStandardOffset=0  TranslationStandardOffsetUnits=m  TranslationROffset=0  TranslationROffsetUnits=m  TranslationThetaOffset=0  TranslationThetaOffsetUnits=deg  TranslationZOffset=0  TranslationZOffsetUnits=m
  z-down : sm_lib/Frames and Transforms/Rigid Transform  RotationMethod=StandardAxis  FollAlignAxisA=+X  BaseAlignAxisA=+Y  FollAlignAxisB=+Y  BaseAlignAxisB=+Z  RotationStandardAxis=+X  RotationAngle=180  RotationAngleUnits=deg  RotationArbitraryAxis=[0 0 1]  RotationSequenceAxes=FollowerAxes  RotationSequence=XYX  RotationSequenceAngles=[0 0 0]  RotationSequenceAnglesUnits=deg  RotationMatrix=[1 0 0; 0 1 0; 0 0 1]  Quaternion=[1 0 0 0]  TranslationMethod=None  TranslationCartesianOffset=[0 0 0]  TranslationCartesianOffsetUnits=m  TranslationStandardAxis=+Z  TranslationStandardOffset=0  TranslationStandardOffsetUnits=m  TranslationROffset=0  TranslationROffsetUnits=m  TranslationThetaOffset=0  TranslationThetaOffsetUnits=deg  TranslationZOffset=0  TranslationZOffsetUnits=m
  Conn1 : PMIOPort  Side=Right
  Conn2 : PMIOPort  Port=2  Side=Left
  connections:
  Conn1/RConn1 -- z-down/RConn1
  y -90/RConn1 -- x +90/LConn1
  x +90/RConn1 -- z-down/LConn1
  Conn2/RConn1 -- y -90/LConn1

== system Crazyflie_Sim_R2025b/6dof joint/Drone Reference Frame z-down,  X  ==
  45deg : sm_lib/Frames and Transforms/Rigid Transform  RotationMethod=StandardAxis  FollAlignAxisA=+X  BaseAlignAxisA=+Y  FollAlignAxisB=+Y  BaseAlignAxisB=+Z  RotationStandardAxis=+Z  RotationAngle=45  RotationAngleUnits=deg  RotationArbitraryAxis=[0 0 1]  RotationSequenceAxes=FollowerAxes  RotationSequence=XYX  RotationSequenceAngles=[0 0 0]  RotationSequenceAnglesUnits=deg  RotationMatrix=[1 0 0; 0 1 0; 0 0 1]  Quaternion=[1 0 0 0]  TranslationMethod=None  TranslationCartesianOffset=[0 0 0]  TranslationCartesianOffsetUnits=m  TranslationStandardAxis=+Z  TranslationStandardOffset=0  TranslationStandardOffsetUnits=m  TranslationROffset=0  TranslationROffsetUnits=m  TranslationThetaOffset=0  TranslationThetaOffsetUnits=deg  TranslationZOffset=0  TranslationZOffsetUnits=m
  x +90 : sm_lib/Frames and Transforms/Rigid Transform  RotationMethod=StandardAxis  FollAlignAxisA=+X  BaseAlignAxisA=+Y  FollAlignAxisB=+Y  BaseAlignAxisB=+Z  RotationStandardAxis=+X  RotationAngle=90  RotationAngleUnits=deg  RotationArbitraryAxis=[0 0 1]  RotationSequenceAxes=FollowerAxes  RotationSequence=XYX  RotationSequenceAngles=[0 0 0]  RotationSequenceAnglesUnits=deg  RotationMatrix=[1 0 0; 0 1 0; 0 0 1]  Quaternion=[1 0 0 0]  TranslationMethod=None  TranslationCartesianOffset=[0 0 0]  TranslationCartesianOffsetUnits=m  TranslationStandardAxis=+Z  TranslationStandardOffset=0  TranslationStandardOffsetUnits=m  TranslationROffset=0  TranslationROffsetUnits=m  TranslationThetaOffset=0  TranslationThetaOffsetUnits=deg  TranslationZOffset=0  TranslationZOffsetUnits=m
  y -90 : sm_lib/Frames and Transforms/Rigid Transform  RotationMethod=StandardAxis  FollAlignAxisA=+X  BaseAlignAxisA=+Y  FollAlignAxisB=+Y  BaseAlignAxisB=+Z  RotationStandardAxis=+Y  RotationAngle=-90  RotationAngleUnits=deg  RotationArbitraryAxis=[0 0 1]  RotationSequenceAxes=FollowerAxes  RotationSequence=XYX  RotationSequenceAngles=[0 0 0]  RotationSequenceAnglesUnits=deg  RotationMatrix=[1 0 0; 0 1 0; 0 0 1]  Quaternion=[1 0 0 0]  TranslationMethod=None  TranslationCartesianOffset=[0 0 0]  TranslationCartesianOffsetUnits=m  TranslationStandardAxis=+Z  TranslationStandardOffset=0  TranslationStandardOffsetUnits=m  TranslationROffset=0  TranslationROffsetUnits=m  TranslationThetaOffset=0  TranslationThetaOffsetUnits=deg  TranslationZOffset=0  TranslationZOffsetUnits=m
  z-down : sm_lib/Frames and Transforms/Rigid Transform  RotationMethod=StandardAxis  FollAlignAxisA=+X  BaseAlignAxisA=+Y  FollAlignAxisB=+Y  BaseAlignAxisB=+Z  RotationStandardAxis=+X  RotationAngle=180  RotationAngleUnits=deg  RotationArbitraryAxis=[0 0 1]  RotationSequenceAxes=FollowerAxes  RotationSequence=XYX  RotationSequenceAngles=[0 0 0]  RotationSequenceAnglesUnits=deg  RotationMatrix=[1 0 0; 0 1 0; 0 0 1]  Quaternion=[1 0 0 0]  TranslationMethod=None  TranslationCartesianOffset=[0 0 0]  TranslationCartesianOffsetUnits=m  TranslationStandardAxis=+Z  TranslationStandardOffset=0  TranslationStandardOffsetUnits=m  TranslationROffset=0  TranslationROffsetUnits=m  TranslationThetaOffset=0  TranslationThetaOffsetUnits=deg  TranslationZOffset=0  TranslationZOffsetUnits=m
  Conn1 : PMIOPort  Side=Right
  Conn2 : PMIOPort  Port=2  Side=Left
  connections:
  Conn2/RConn1 -- y -90/LConn1
  x +90/RConn1 -- z-down/LConn1
  y -90/RConn1 -- x +90/LConn1
  z-down/RConn1 -- 45deg/LConn1
  45deg/RConn1 -- Conn1/RConn1

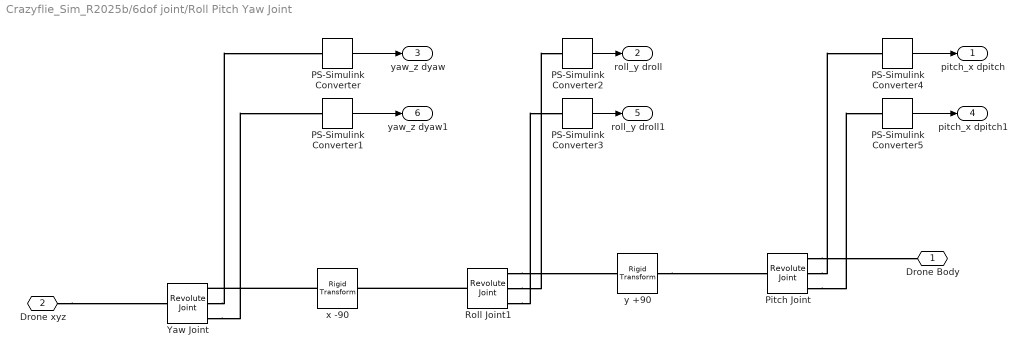
== system Crazyflie_Sim_R2025b/6dof joint/Roll Pitch Yaw Joint ==
  PS-Simulink Converter{,1..5} (6 alike) : nesl_utility/PS-Simulink Converter  PhysicalDomain=network_engine_domain  SubClassName=ps_output  LeftPortType=input  RightPortType=output  PseudoPeriodic=off  Frequencies=[]  VectorFormat=1-D array  Unit=1  AffineConversion=off
  Pitch Joint : sm_lib/Joints/Revolute Joint  JointMode=Normal  CompositeWrenchDir=FollowerOnBase  CompositeWrenchFrame=BaseFrame  SenseConstraintForce=off  SenseConstraintTorque=off  SenseTotalForce=off  SenseTotalTorque=off  PositionTargetSpecify=off  PositionTargetPriority=High  PositionTargetValue=0  PositionTargetValueUnits=deg  VelocityTargetSpecify=off  VelocityTargetPriority=High  VelocityTargetValue=0  VelocityTargetValueUnits=deg/s  EquilibriumPosition=0  EquilibriumPositionUnits=deg  SpringStiffness=0  SpringStiffnessUnits=N*m/deg  DampingCoefficient=0  DampingCoefficientUnits=N*m/(deg/s)  LowerLimitSpecify=off  LowerLimitBound=-90  LowerLimitBoundUnits=deg  LowerLimitStiffness=1e4  LowerLimitStiffnessUnits=N*m/deg  LowerLimitDamping=10  LowerLimitDampingUnits=N*m/(deg/s)  LowerLimitTransitionRegionWidth=0.1  LowerLimitTransitionRegionWidthUnits=deg  UpperLimitSpecify=off  UpperLimitBound=90  UpperLimitBoundUnits=deg  UpperLimitStiffness=1e4  UpperLimitStiffnessUnits=N*m/deg  UpperLimitDamping=10  UpperLimitDampingUnits=N*m/(deg/s)  UpperLimitTransitionRegionWidth=0.1  UpperLimitTransitionRegionWidthUnits=deg  TorqueActuationMode=NoTorque  MotionActuationMode=ComputedMotion  SensePosition=on  SenseVelocity=on  SenseAcceleration=off  SenseTorqueForce=off  SenseLowerLimitTorqueForce=off  SenseUpperLimitTorqueForce=off
  Roll Joint1 : sm_lib/Joints/Revolute Joint  JointMode=Normal  CompositeWrenchDir=FollowerOnBase  CompositeWrenchFrame=BaseFrame  SenseConstraintForce=off  SenseConstraintTorque=off  SenseTotalForce=off  SenseTotalTorque=off  PositionTargetSpecify=off  PositionTargetPriority=High  PositionTargetValue=0  PositionTargetValueUnits=deg  VelocityTargetSpecify=off  VelocityTargetPriority=High  VelocityTargetValue=0  VelocityTargetValueUnits=deg/s  EquilibriumPosition=0  EquilibriumPositionUnits=deg  SpringStiffness=0  SpringStiffnessUnits=N*m/deg  DampingCoefficient=0  DampingCoefficientUnits=N*m/(deg/s)  LowerLimitSpecify=off  LowerLimitBound=-90  LowerLimitBoundUnits=deg  LowerLimitStiffness=1e4  LowerLimitStiffnessUnits=N*m/deg  LowerLimitDamping=10  LowerLimitDampingUnits=N*m/(deg/s)  LowerLimitTransitionRegionWidth=0.1  LowerLimitTransitionRegionWidthUnits=deg  UpperLimitSpecify=off  UpperLimitBound=90  UpperLimitBoundUnits=deg  UpperLimitStiffness=1e4  UpperLimitStiffnessUnits=N*m/deg  UpperLimitDamping=10  UpperLimitDampingUnits=N*m/(deg/s)  UpperLimitTransitionRegionWidth=0.1  UpperLimitTransitionRegionWidthUnits=deg  TorqueActuationMode=NoTorque  MotionActuationMode=ComputedMotion  SensePosition=on  SenseVelocity=on  SenseAcceleration=off  SenseTorqueForce=off  SenseLowerLimitTorqueForce=off  SenseUpperLimitTorqueForce=off
  Yaw Joint : sm_lib/Joints/Revolute Joint  JointMode=Normal  CompositeWrenchDir=FollowerOnBase  CompositeWrenchFrame=BaseFrame  SenseConstraintForce=off  SenseConstraintTorque=off  SenseTotalForce=off  SenseTotalTorque=off  PositionTargetSpecify=off  PositionTargetPriority=High  PositionTargetValue=0  PositionTargetValueUnits=deg  VelocityTargetSpecify=off  VelocityTargetPriority=High  VelocityTargetValue=0  VelocityTargetValueUnits=deg/s  EquilibriumPosition=0  EquilibriumPositionUnits=deg  SpringStiffness=0  SpringStiffnessUnits=N*m/deg  DampingCoefficient=0  DampingCoefficientUnits=N*m/(deg/s)  LowerLimitSpecify=off  LowerLimitBound=-90  LowerLimitBoundUnits=deg  LowerLimitStiffness=1e4  LowerLimitStiffnessUnits=N*m/deg  LowerLimitDamping=10  LowerLimitDampingUnits=N*m/(deg/s)  LowerLimitTransitionRegionWidth=0.1  LowerLimitTransitionRegionWidthUnits=deg  UpperLimitSpecify=off  UpperLimitBound=90  UpperLimitBoundUnits=deg  UpperLimitStiffness=1e4  UpperLimitStiffnessUnits=N*m/deg  UpperLimitDamping=10  UpperLimitDampingUnits=N*m/(deg/s)  UpperLimitTransitionRegionWidth=0.1  UpperLimitTransitionRegionWidthUnits=deg  TorqueActuationMode=NoTorque  MotionActuationMode=ComputedMotion  SensePosition=on  SenseVelocity=on  SenseAcceleration=off  SenseTorqueForce=off  SenseLowerLimitTorqueForce=off  SenseUpperLimitTorqueForce=off
  x -90 : sm_lib/Frames and Transforms/Rigid Transform  RotationMethod=StandardAxis  FollAlignAxisA=+X  BaseAlignAxisA=+Y  FollAlignAxisB=+Y  BaseAlignAxisB=+Z  RotationStandardAxis=+X  RotationAngle=-90  RotationAngleUnits=deg  RotationArbitraryAxis=[0 0 1]  RotationSequenceAxes=FollowerAxes  RotationSequence=XYX  RotationSequenceAngles=[0 0 0]  RotationSequenceAnglesUnits=deg  RotationMatrix=[1 0 0; 0 1 0; 0 0 1]  Quaternion=[1 0 0 0]  TranslationMethod=None  TranslationCartesianOffset=[0 0 0]  TranslationCartesianOffsetUnits=m  TranslationStandardAxis=+Z  TranslationStandardOffset=0  TranslationStandardOffsetUnits=m  TranslationROffset=0  TranslationROffsetUnits=m  TranslationThetaOffset=0  TranslationThetaOffsetUnits=deg  TranslationZOffset=0  TranslationZOffsetUnits=m
  y +90 : sm_lib/Frames and Transforms/Rigid Transform  RotationMethod=StandardAxis  FollAlignAxisA=+X  BaseAlignAxisA=+Y  FollAlignAxisB=+Y  BaseAlignAxisB=+Z  RotationStandardAxis=+Y  RotationAngle=90  RotationAngleUnits=deg  RotationArbitraryAxis=[0 0 1]  RotationSequenceAxes=FollowerAxes  RotationSequence=XYX  RotationSequenceAngles=[0 0 0]  RotationSequenceAnglesUnits=deg  RotationMatrix=[1 0 0; 0 1 0; 0 0 1]  Quaternion=[1 0 0 0]  TranslationMethod=None  TranslationCartesianOffset=[0 0 0]  TranslationCartesianOffsetUnits=m  TranslationStandardAxis=+Z  TranslationStandardOffset=0  TranslationStandardOffsetUnits=m  TranslationROffset=0  TranslationROffsetUnits=m  TranslationThetaOffset=0  TranslationThetaOffsetUnits=deg  TranslationZOffset=0  TranslationZOffsetUnits=m
  Drone Body : PMIOPort  Side=Right
  Drone xyz : PMIOPort  Port=2  Side=Left
  pitch_x dpitch : Outport
  roll_y droll : Outport  Port=2
  yaw_z dyaw : Outport  Port=3
  pitch_x dpitch1 : Outport  Port=4
  roll_y droll1 : Outport  Port=5
  yaw_z dyaw1 : Outport  Port=6
  wires:
  PS-Simulink Converter2/1 -> roll_y droll/1
  PS-Simulink Converter5/1 -> pitch_x dpitch1/1
  PS-Simulink Converter/1 -> yaw_z dyaw/1
  PS-Simulink Converter1/1 -> yaw_z dyaw1/1
  PS-Simulink Converter4/1 -> pitch_x dpitch/1
  PS-Simulink Converter3/1 -> roll_y droll1/1
  connections:
  Drone xyz/RConn1 -- Yaw Joint/LConn1
  x -90/LConn1 -- Yaw Joint/RConn1
  Pitch Joint/RConn1 -- Drone Body/RConn1
  Roll Joint1/LConn1 -- x -90/RConn1
  y +90/RConn1 -- Pitch Joint/LConn1
  Pitch Joint/RConn2 -- PS-Simulink Converter4/LConn1
  Yaw Joint/RConn2 -- PS-Simulink Converter/LConn1
  Roll Joint1/RConn2 -- PS-Simulink Converter2/LConn1
  Roll Joint1/RConn3 -- PS-Simulink Converter3/LConn1
  Yaw Joint/RConn3 -- PS-Simulink Converter1/LConn1
  Pitch Joint/RConn3 -- PS-Simulink Converter5/LConn1
  Roll Joint1/RConn1 -- y +90/LConn1
